simulink model "TCC_FV_BESS_R2023"  (R2023b)
settings: Solver=ode23tb  StartTime=0.0  StopTime=86400  MaxStep=60  RelTol=1e-3  AbsTol=1e-4
settings Model: Creator=LUAN  LastModifiedBy=LUAN

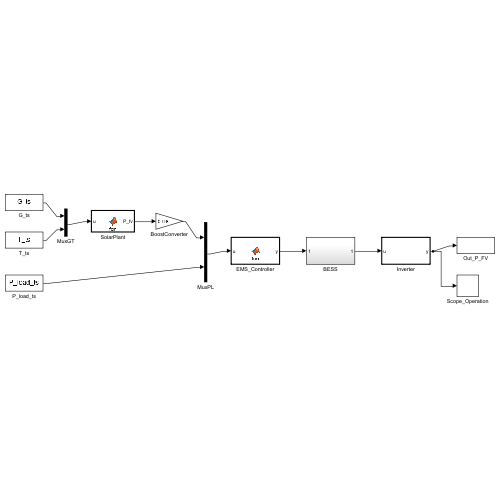
[thumbnail: Simulink's stored preview of the top-level diagram]
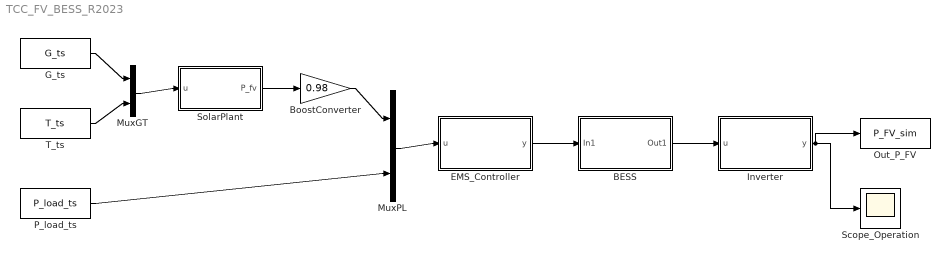
== system TCC_FV_BESS_R2023 ==
  BESS : Subsystem
  BoostConverter : Gain  Gain=0.98
  EMS_Controller : MATLAB Function  TreatAsAtomicUnit=on
  G_ts : FromWorkspace  VariableName=G_ts  OutputAfterFinalValue=Holding final value
  Inverter : MATLAB Function  TreatAsAtomicUnit=on
  MuxGT : Mux  Inputs=2
  MuxPL : Mux  Inputs=2
  Out_P_FV : ToWorkspace  VariableName=P_FV_sim  SaveFormat=Structure With Time  SampleTime=60
  P_load_ts : FromWorkspace  VariableName=P_load_ts  OutputAfterFinalValue=Holding final value
  Scope_Operation : Scope
  SolarPlant : MATLAB Function  TreatAsAtomicUnit=on
  T_ts : FromWorkspace  VariableName=T_ts  OutputAfterFinalValue=Holding final value
  wires:
  G_ts/1 -> MuxGT/1
  T_ts/1 -> MuxGT/2
  MuxGT/1 -> SolarPlant/1(u)
  SolarPlant/1(P_fv) -> BoostConverter/1
  BoostConverter/1 -> MuxPL/1
  P_load_ts/1 -> MuxPL/2
  MuxPL/1 -> EMS_Controller/1(u)
  EMS_Controller/1(y) -> BESS/1(In1)
  BESS/1(Out1) -> Inverter/1(u)
  Inverter/1(y) -> Out_P_FV/1, Scope_Operation/1

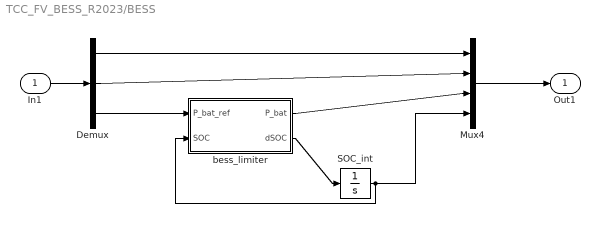
== system TCC_FV_BESS_R2023/BESS ==
  In1 : Inport
  Demux : Demux  Outputs=3
  Mux4 : Mux
  SOC_int : Integrator  InitialCondition=50  LimitOutput=on  UpperSaturationLimit=90  LowerSaturationLimit=20
  bess_limiter : MATLAB Function  TreatAsAtomicUnit=on
  Out1 : Outport
  wires:
  In1/1 -> Demux/1
  Demux/1 -> Mux4/1
  Demux/2 -> Mux4/2
  Demux/3 -> bess_limiter/1(P_bat_ref)
  bess_limiter/1(P_bat) -> Mux4/3
  bess_limiter/2(dSOC) -> SOC_int/1
  SOC_int/1 -> bess_limiter/2(SOC), Mux4/4
  Mux4/1 -> Out1/1

== matlab function TCC_FV_BESS_R2023/SolarPlant ==
  data: u input; P_fv output
function P_fv = fcn(u)
% SolarPlant — Eq. 05 do TCC (potência corrigida por temperatura)
G = u(1); T = u(2);
T_cel = T + (45-20)/800*G;                % modelo NOCT
P_fv  = 5000*(G/1000)*(1 - 0.004*(T_cel-25));
P_fv  = max(P_fv, 0);

== matlab function TCC_FV_BESS_R2023/BESS/bess_limiter ==
  data: P_bat_ref input; P_bat output; SOC input; dSOC output
function [P_bat, dSOC] = fcn(P_bat_ref, SOC)
% BESS — Eq. 16/17 (Coulomb counting em base energética) + janela SOC
if P_bat_ref > 0 && SOC < 90
    P_bat = min(P_bat_ref, 5000);
    dSOC  = 100*0.96*P_bat/3.6e+07;           % [%/s]
elseif P_bat_ref < 0 && SOC > 20
    P_bat = max(P_bat_ref, -5000);
    dSOC  = 100*P_bat/(0.96*3.6e+07);
else
    P_bat = 0; dSOC = 0;
end

== matlab function TCC_FV_BESS_R2023/Inverter ==
  data: u input; y output
function y = fcn(u)
% Inverter — Eq. 18/21/23 (balanço com a rede)
P_dc = u(1); P_load = u(2); P_bat = u(3); SOC = u(4);
P_ac   = 0.97*(P_dc - P_bat);              % CC liquido -> CA
P_grid = P_load - P_ac;                    % >0 importa, <0 exporta
y = [P_dc; P_load; P_bat; SOC; P_grid];

== matlab function TCC_FV_BESS_R2023/EMS_Controller ==
  data: u input; y output
function y = fcn(u)
% EMS_Controller — regras da FIGURA 04 (referência pelo saldo)
P_dc = u(1); P_load = u(2);
saldo = P_dc - P_load;
if saldo > 0
    P_bat_ref = min(saldo, 5000);          % pedido de carga
else
    P_bat_ref = -min(-saldo, 5000);        % pedido de descarga
end
y = [P_dc; P_load; P_bat_ref];
